simulink model "XCOMM01_reference"  (R2025a)
settings: Solver=FixedStepDiscrete  StartTime=0  StopTime=0.16  FixedStep=1.0000000000000001e-05  RelTol=1e-3
undefined symbols (not defined in the file): clutter_ratio, interference_duration, interference_ratio, interference_time, snr_db, target1_range, target1_rcs, target1_velocity, target2_range, target2_rcs, target2_velocity
settings Model: Creator=SimuVerity Contributors  LastModifiedBy=SimuVerity Contributors

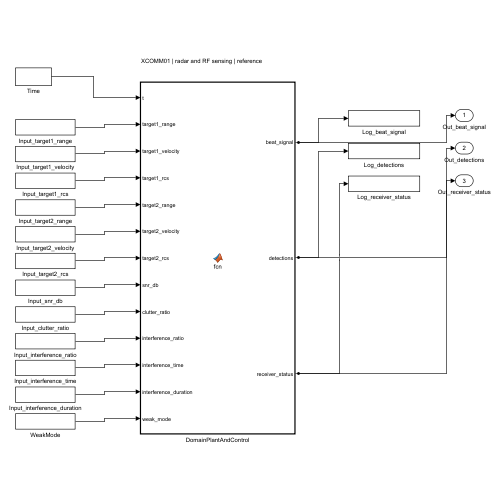
[thumbnail: Simulink's stored preview of the top-level diagram]
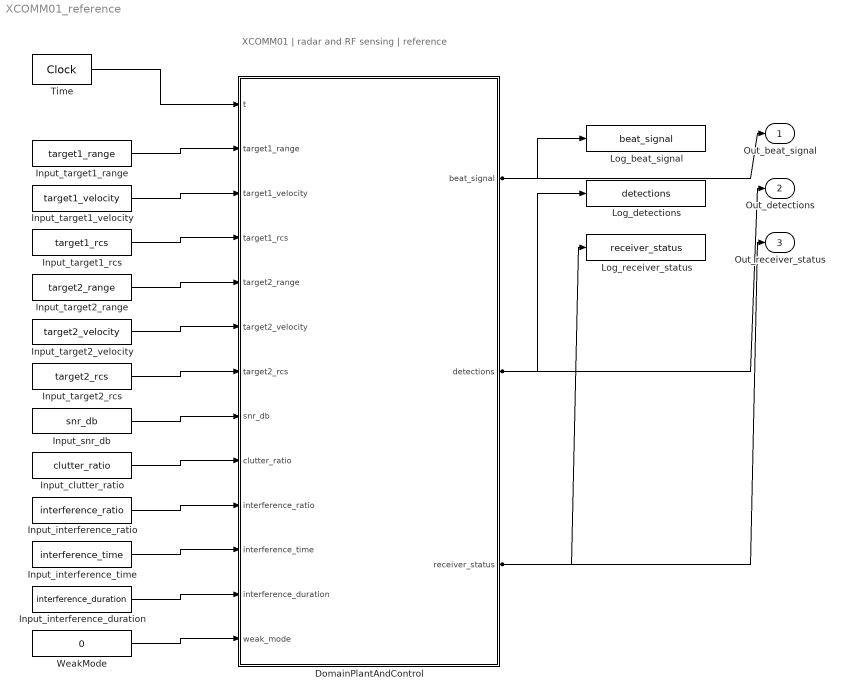
== system XCOMM01_reference ==
  note: XCOMM01 | radar and RF sensing | reference
  DomainPlantAndControl : MATLAB Function  TreatAsAtomicUnit=on
  Input_clutter_ratio : Constant  Value=clutter_ratio
  Input_interference_duration : Constant  Value=interference_duration
  Input_interference_ratio : Constant  Value=interference_ratio
  Input_interference_time : Constant  Value=interference_time
  Input_snr_db : Constant  Value=snr_db
  Input_target1_range : Constant  Value=target1_range
  Input_target1_rcs : Constant  Value=target1_rcs
  Input_target1_velocity : Constant  Value=target1_velocity
  Input_target2_range : Constant  Value=target2_range
  Input_target2_rcs : Constant  Value=target2_rcs
  Input_target2_velocity : Constant  Value=target2_velocity
  Log_beat_signal : ToWorkspace  VariableName=beat_signal  SaveFormat=Timeseries  SampleTime=-1
  Log_detections : ToWorkspace  VariableName=detections  SaveFormat=Timeseries  SampleTime=-1
  Log_receiver_status : ToWorkspace  VariableName=receiver_status  SaveFormat=Timeseries  SampleTime=-1
  Time : DigitalClock  SampleTime=1.0000000000000001e-05
  WeakMode : Constant  Value=0
  Out_beat_signal : Outport
  Out_detections : Outport  Port=2
  Out_receiver_status : Outport  Port=3
  wires:
  Time/1 -> DomainPlantAndControl/1(t)
  Input_target1_range/1 -> DomainPlantAndControl/2(target1_range)
  Input_target1_velocity/1 -> DomainPlantAndControl/3(target1_velocity)
  Input_target1_rcs/1 -> DomainPlantAndControl/4(target1_rcs)
  Input_target2_range/1 -> DomainPlantAndControl/5(target2_range)
  Input_target2_velocity/1 -> DomainPlantAndControl/6(target2_velocity)
  Input_target2_rcs/1 -> DomainPlantAndControl/7(target2_rcs)
  Input_snr_db/1 -> DomainPlantAndControl/8(snr_db)
  Input_clutter_ratio/1 -> DomainPlantAndControl/9(clutter_ratio)
  Input_interference_ratio/1 -> DomainPlantAndControl/10(interference_ratio)
  Input_interference_time/1 -> DomainPlantAndControl/11(interference_time)
  Input_interference_duration/1 -> DomainPlantAndControl/12(interference_duration)
  WeakMode/1 -> DomainPlantAndControl/13(weak_mode)
  DomainPlantAndControl/1(beat_signal) -> Log_beat_signal/1, Out_beat_signal/1
  DomainPlantAndControl/2(detections) -> Log_detections/1, Out_detections/1
  DomainPlantAndControl/3(receiver_status) -> Log_receiver_status/1, Out_receiver_status/1

== matlab function XCOMM01_reference/DomainPlantAndControl ==
  data: t input; beat_signal output; target1_range input; target1_velocity input; target1_rcs input; target2_range input; target2_velocity input; target2_rcs input; snr_db input; clutter_ratio input; interference_ratio input; interference_time input; interference_duration input; weak_mode input; detections output; receiver_status output
function [beat_signal,detections,receiver_status] = fcn(t,target1_range,target1_velocity,target1_rcs,target2_range,target2_velocity,target2_rcs,snr_db,clutter_ratio,interference_ratio,interference_time,interference_duration,weak_mode)
%#codegen
persistent r1h r2h v1h v2h c1 c2 lock fa sampleIndex chirpIndex sampleBuffer upSpectrum downSpectrum haveUp jamBandBaseUp jamBandBaseDown energyBaseUp energyBaseDown jamFlag baseConf
dt=1e-5; c0=299792458; fc=77e9; slope=3.5e10; T=0.004; N=400; Fs=1/dt;
if isempty(r1h) || t<0.5*dt
    r1h=48; r2h=103; v1h=0; v2h=0; c1=.12; c2=.10; lock=.08; fa=.22;
    sampleIndex=1; chirpIndex=0; sampleBuffer=complex(zeros(1,N)); upSpectrum=zeros(1,N); downSpectrum=zeros(1,N);
    haveUp=false; jamBandBaseUp=0; jamBandBaseDown=0; energyBaseUp=0; energyBaseDown=0; jamFlag=0; baseConf=.12;
end
tc=mod(t,T); chirpDirection=1-2*mod(floor(t/T),2);
fb1=2*slope*target1_range/c0; fb2=2*slope*target2_range/c0;
fd1=2*target1_velocity*fc/c0; fd2=2*target2_velocity*fc/c0;
a1=sqrt(max(target1_rcs,.1))/(target1_range/50)^2; a2=sqrt(max(target2_rcs,.1))/(target2_range/50)^2; asum=a1+a2;
slowTime=floor(t/T)*T;
ph1=2*pi*((chirpDirection*fb1+fd1)*tc+fd1*slowTime);
ph2=2*pi*((chirpDirection*fb2+fd2)*tc+fd2*slowTime);
targetI=a1*cos(ph1)+a2*cos(ph2); targetQ=a1*sin(ph1)+a2*sin(ph2);
clutter=clutter_ratio*asum; clutterPhase=2*pi*(chirpDirection*1850)*tc; clutterI=clutter*cos(clutterPhase); clutterQ=clutter*sin(clutterPhase);
noiseAmp=asum*10^(-snr_db/20); noiseI=noiseAmp*(.66*sin(2*pi*31415*t)+.34*sin(2*pi*27183*t));
noiseQ=noiseAmp*(.61*cos(2*pi*29611*t)+.39*sin(2*pi*22307*t));
event=(t>=interference_time && t<interference_time+interference_duration); jam=interference_ratio*asum*double(event);
jamI=jam*cos(2*pi*37100*t+.3); jamQ=jam*sin(2*pi*37100*t+.3);
measI=targetI+clutterI+noiseI+jamI; measQ=targetQ+clutterQ+noiseQ+jamQ;
sampleBuffer(sampleIndex)=complex(measI,measQ);
if sampleIndex>=N
    spectrum=abs(fft(sampleBuffer));
    jamLevel=jam_band_energy(spectrum,Fs); energyLevel=sum(spectrum.^2);
    if mod(chirpIndex,2)==0
        if jamBandBaseUp<=0, jamBandBaseUp=max(jamLevel,eps); energyBaseUp=max(energyLevel,eps); end
        if chirpIndex<6, jamFlag=0; else, jamFlag=double(jamLevel>2.5*jamBandBaseUp || energyLevel>1.025*energyBaseUp); end
        if jamFlag<.5, jamBandBaseUp=max(.998*jamBandBaseUp,jamLevel); energyBaseUp=max(.998*energyBaseUp,energyLevel); end
        upSpectrum=spectrum; haveUp=true;
    else
        if jamBandBaseDown<=0, jamBandBaseDown=max(jamLevel,eps); energyBaseDown=max(energyLevel,eps); end
        if chirpIndex<6, jamFlag=0; else, jamFlag=double(jamLevel>2.5*jamBandBaseDown || energyLevel>1.025*energyBaseDown); end
        if jamFlag<.5, jamBandBaseDown=max(.998*jamBandBaseDown,jamLevel); energyBaseDown=max(.998*energyBaseDown,energyLevel); end
        downSpectrum=spectrum;
        if haveUp
            [fu,au]=peak_list(upSpectrum,Fs); [fd,ad]=peak_list(downSpectrum,Fs);
            [rn,vn,sn]=estimate_band(fu,au,fd,ad,35,78);
            [rf,vf,sf]=estimate_band(fu,au,fd,ad,78,130);
            quality=min(sn,sf)/max((sum(upSpectrum)+sum(downSpectrum))/(2*N),eps);
            baseConf=clamp01((quality-1.4)/3.5);
            if sn>0 && sf>0 && jamFlag<.5
                if weak_mode<.5
                    alpha=.82; g1=rn; g2=rf; h1=vn; h2=vf;
                else
                    alpha=.28; g1=.84*rn+11; g2=.82*rf+13; h1=.12*vn; h2=.10*vf; baseConf=min(baseConf,.62);
                end
                r1h=r1h+alpha*(g1-r1h); r2h=r2h+alpha*(g2-r2h); v1h=v1h+alpha*(h1-v1h); v2h=v2h+alpha*(h2-v2h);
            end
        end
    end
    sampleIndex=1; chirpIndex=chirpIndex+1; sampleBuffer(:)=0;
else
    sampleIndex=sampleIndex+1;
end
confGoal=baseConf; if jamFlag>.5, confGoal=min(confGoal,.24); end
if weak_mode>=.5, confGoal=min(confGoal,.60); end
beta=min(dt/.0015,1); c1=c1+beta*(confGoal-c1); c2=c2+beta*(max(confGoal-.025,0)-c2);
lockGoal=clamp01(1.02*confGoal); faGoal=clamp01(.004+.16*(1-confGoal)+.18*jamFlag);
lock=lock+beta*(lockGoal-lock); fa=fa+beta*(faGoal-fa);
beat_signal=[measI,measQ];
detections=[r1h,v1h,min(max(c1,0),1),r2h,v2h,min(max(c2,0),1)];
receiver_status=[min(max(lock,0),1),min(max(fa,0),1),jamFlag];
end

function [freq,amp]=peak_list(mag,Fs)
N=400; K=10; work=mag; freq=zeros(1,K); amp=zeros(1,K);
work(1)=0; work(N/2+1)=0;
for p=1:K
    [amp(p),idx]=max(work); delta=0;
    if idx>1 && idx<N
        yl=log(max(mag(idx-1),eps)); yc=log(max(mag(idx),eps)); yr=log(max(mag(idx+1),eps)); den=yl-2*yc+yr;
        if abs(den)>1e-12, delta=max(min(.5*(yl-yr)/den,.5),-.5); end
    end
    bin=(idx-1)+delta; if bin>N/2, bin=bin-N; end; freq(p)=bin*Fs/N;
    lo=max(1,idx-1); hi=min(N,idx+1); work(lo:hi)=0;
end
end

function [bestR,bestV,bestStrength]=estimate_band(fu,au,fd,ad,rlo,rhi)
c0=299792458; fc=77e9; slope=3.5e10; bestR=(rlo+rhi)/2; bestV=0; bestStrength=0;
for i=1:10
    for j=1:10
        rr=(fu(i)-fd(j))*c0/(4*slope); vv=(fu(i)+fd(j))*c0/(4*fc);
        if rr>=rlo && rr<=rhi && vv>=-23 && vv<=21
            balance=min(au(i),ad(j))/max(max(au(i),ad(j)),eps); strength=min(au(i),ad(j))*sqrt(balance);
            if strength>bestStrength, bestStrength=strength; bestR=rr; bestV=vv; end
        end
    end
end
end

function e=jam_band_energy(mag,Fs)
N=400; e=0;
for k=1:N
    bin=k-1; if bin>N/2, bin=bin-N; end; f=bin*Fs/N;
    if abs(f-37100)<=900, e=e+mag(k); end
end
end

function y=clamp01(x)
y=min(max(x,0),1);
end
